simulink model "TEST"  (R2023a)
settings: Solver=ode1  StartTime=0.0  StopTime=tsim  FixedStep=CONTROL.Tm  RelTol=1e-3
undefined symbols (not defined in the file): Bm, J, MOTOR, tfalta, Tload, wini
libraries: simulink x2
settings Model: Creator=Usuario  LastModifiedBy=Usuario
settings DataIOCC: ReturnWorkspaceOutputs=off  TimeSaveName=time

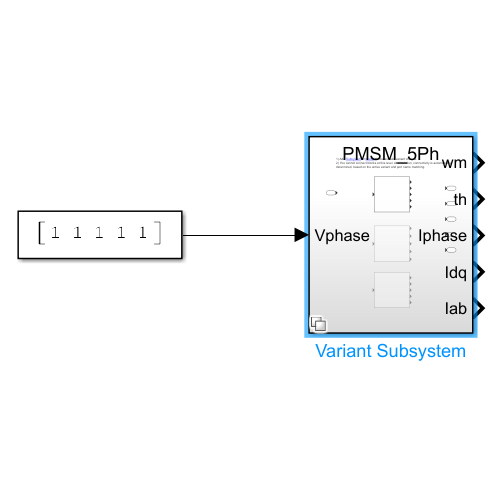
[thumbnail: Simulink's stored preview of the top-level diagram]
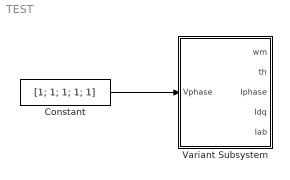
== system TEST ==
  Constant : Constant  Value=[1; 1; 1; 1; 1]
  Variant Subsystem : Subsystem  Variant=on
  wires:
  Constant/1 -> Variant Subsystem/1(Vphase)

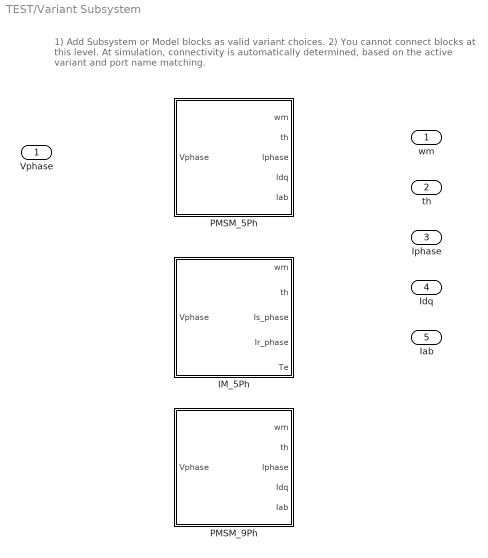
== system TEST/Variant Subsystem ==
  note: 1) Add Subsystem or Model blocks as valid variant choices.
      | 2) You cannot connect blocks at this level. At simulation, connectivity is automatically
      | determined, based on the active variant and port name matching.
  Vphase : Inport
  IM_5Ph : Subsystem  VariantControl=MOTOR.Index == 2
  PMSM_5Ph : Subsystem  VariantControl=MOTOR.Index == 1
  PMSM_9Ph : Subsystem  VariantControl=MOTOR.Index == 3
  wm : Outport
  th : Outport  Port=2
  Iphase : Outport  Port=3
  Idq : Outport  Port=4
  Iab : Outport  Port=5

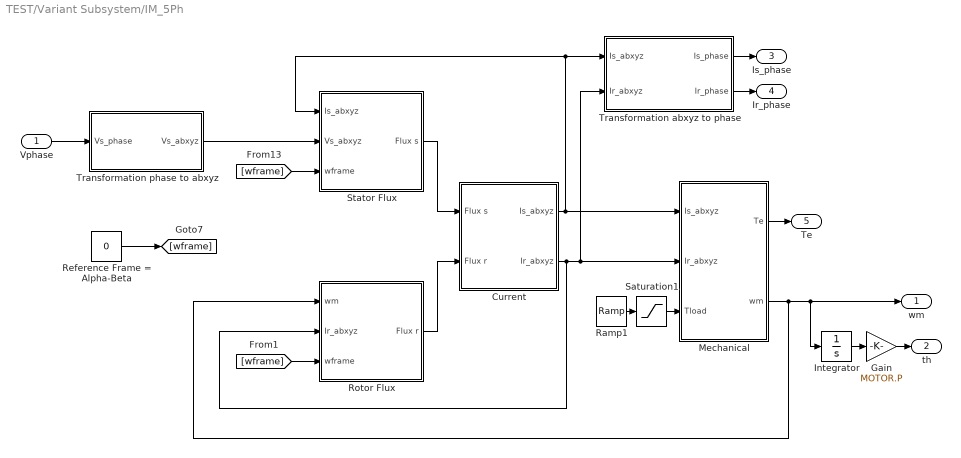
== system TEST/Variant Subsystem/IM_5Ph ==
  Vphase : Inport
  Current : Subsystem
  Gain : Gain  Gain=MOTOR.P
  Integrator : Integrator
  Mechanical : Subsystem
  Ramp1 : simulink/Sources/Ramp  slope=40*Tload  start=0  InitialOutput=0
  Reference Frame = Alpha-Beta : Constant  Value=0
  Rotor Flux : Subsystem
  Saturation1 : Saturate  UpperLimit=Tload  LowerLimit=0
  "Stator Flux " : Subsystem
  Transformation abxyz to phase : Subsystem
  Transformation phase to abxyz : Subsystem
  wm : Outport  VectorParamsAs1DForOutWhenUnconnected=off
  th : Outport  Port=2  VectorParamsAs1DForOutWhenUnconnected=off
  Is_phase : Outport  Port=3  VectorParamsAs1DForOutWhenUnconnected=off
  Ir_phase : Outport  Port=4  VectorParamsAs1DForOutWhenUnconnected=off
  Te : Outport  Port=5  VectorParamsAs1DForOutWhenUnconnected=off
  wires:
  Mechanical/1(Te) -> Te/1
  Transformation abxyz to phase/2(Ir_phase) -> Ir_phase/1
  [wframe] -> "Stator Flux "/3(wframe)
  Transformation phase to abxyz/1(Vs_abxyz) -> "Stator Flux "/2(Vs_abxyz)
  Ramp1/1 -> Saturation1/1
  Vphase/1 -> Transformation phase to abxyz/1(Vs_phase)
  Current/2(Ir_abxyz) -> Rotor Flux/2(Ir_abxyz), Transformation abxyz to phase/2(Ir_abxyz), Mechanical/2(Ir_abxyz)
  Current/1(Is_abxyz) -> Transformation abxyz to phase/1(Is_abxyz), "Stator Flux "/1(Is_abxyz), Mechanical/1(Is_abxyz)
  "Stator Flux "/1(Flux s) -> Current/1(Flux s)
  Reference Frame = Alpha-Beta/1 -> [wframe]
  Mechanical/2(wm) -> Integrator/1, wm/1, Rotor Flux/1(wm)
  Rotor Flux/1(Flux r) -> Current/2(Flux r)
  [wframe] -> Rotor Flux/3(wframe)
  Saturation1/1 -> Mechanical/3(Tload)
  Transformation abxyz to phase/1(Is_phase) -> Is_phase/1
  Integrator/1 -> Gain/1
  Gain/1 -> th/1

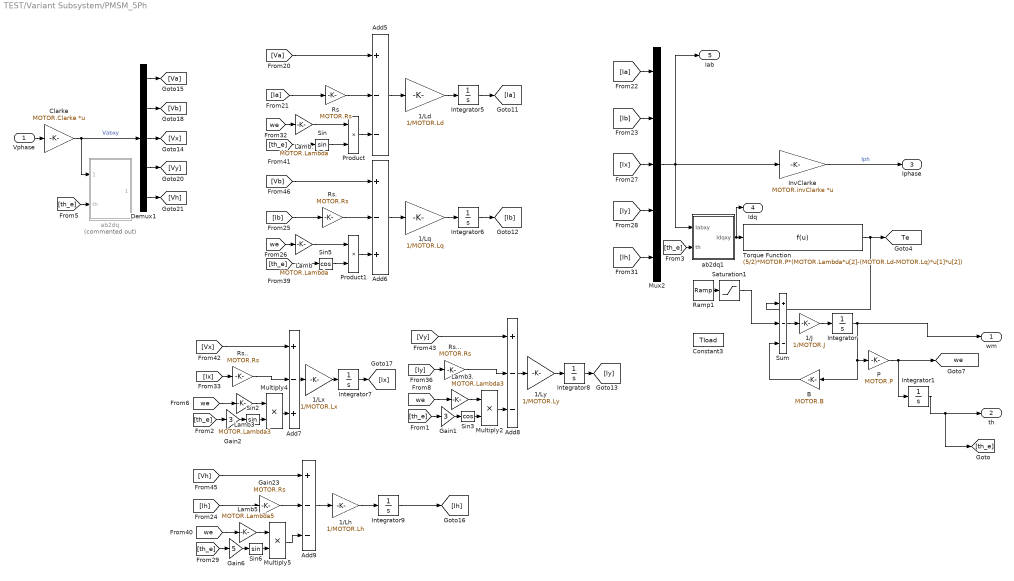
== system TEST/Variant Subsystem/PMSM_5Ph ==
  Vphase : Inport
  1/J : Gain  Gain=1/MOTOR.J
  1/Ld : Gain  Gain=1/MOTOR.Ld
  1/Lh : Gain  Gain=1/MOTOR.Lh
  1/Lq : Gain  Gain=1/MOTOR.Lq
  1/Lx : Gain  Gain=1/MOTOR.Lx
  1/Ly : Gain  Gain=1/MOTOR.Ly
  Add5 : Sum  Inputs=+--
  Add6 : Sum  Inputs=+-+
  Add7 : Sum  Inputs=+-+
  Add8 : Sum  Inputs=+--
  Add9 : Sum  Inputs=+--
  B : Gain  Gain=MOTOR.B
  Clarke : Gain  Gain=MOTOR.Clarke  Multiplication=Matrix(K*u)
  Constant3 : Constant  Value=Tload
  Demux1 : Demux  Outputs=5
  Gain1 : Gain  Gain=3
  Gain2 : Gain  Gain=3
  Gain23 : Gain  Gain=MOTOR.Rs
  Gain6 : Gain  Gain=5
  Integrator{,1,5..9} (7 alike) : Integrator
  InvClarke : Gain  Gain=MOTOR.invClarke  Multiplication=Matrix(K*u)
  Lamb : Gain  Gain=MOTOR.Lambda
  Lamb. : Gain  Gain=MOTOR.Lambda
  Lamb3 : Gain  Gain=MOTOR.Lambda3
  Lamb3. : Gain  Gain=MOTOR.Lambda3
  Lamb5 : Gain  Gain=MOTOR.Lambda5
  Multiply2 : Product
  Multiply4 : Product
  Multiply5 : Product
  Mux2 : Mux  Inputs=5
  P : Gain  Gain=MOTOR.P
  Product : Product
  Product1 : Product
  Ramp1 : simulink/Sources/Ramp  slope=40*Tload  start=0  InitialOutput=0
  Rs : Gain  Gain=MOTOR.Rs
  Rs. : Gain  Gain=MOTOR.Rs
  Rs.. : Gain  Gain=MOTOR.Rs
  Rs... : Gain  Gain=MOTOR.Rs
  Saturation1 : Saturate  UpperLimit=Tload  LowerLimit=0
  Sin : Trigonometry
  Sin2 : Trigonometry
  Sin3 : Trigonometry  Operator=cos
  Sin5 : Trigonometry  Operator=cos
  Sin6 : Trigonometry
  Sum : Sum  Inputs=+--
  Torque Function : Fcn  Expr=(5/2)*MOTOR.P*(MOTOR.Lambda*u[2]-(MOTOR.Ld-MOTOR.Lq)*u[1]*u[2])
  ab2dq : MATLAB Function  Commented=on  TreatAsAtomicUnit=on
  ab2dq1 : MATLAB Function  TreatAsAtomicUnit=on
  wm : Outport
  th : Outport  Port=2
  Iphase : Outport  Port=3
  Idq : Outport  Port=4
  Iab : Outport  Port=5
  tag scope: Te=global, we=global
  wires:
  Gain6/1 -> Sin6/1
  [we] -> Lamb5/1
  Ramp1/1 -> Saturation1/1
  Sin6/1 -> Multiply5/2
  [Va] -> Add5/1
  Lamb5/1 -> Multiply5/1
  Gain1/1 -> Sin3/1
  Lamb3./1 -> Multiply2/1
  1/Lq/1 -> Integrator6/1
  Add8/1 -> 1/Ly/1
  [th_e] -> Gain1/1
  [th_e] -> Gain6/1
  [we] -> Lamb3./1
  Add6/1 -> 1/Lq/1
  [Ix] -> Mux2/3
  Sin/1 -> Product/2
  [th_e] -> Sin/1
  Vphase/1 -> Clarke/1
  1/Ly/1 -> Integrator8/1
  [th_e] -> Sin5/1
  Integrator8/1 -> [Iy]
  Multiply2/1 -> Add8/3
  [we] -> Lamb/1
  Demux1/3 -> [Vx]
  Sin3/1 -> Multiply2/2
  Lamb/1 -> Product1/1
  Sin5/1 -> Product1/2
  ab2dq1/1(Idqxy) -> Torque Function/1, Idq/1
  Rs/1 -> Add5/2
  Rs.../1 -> Add8/2
  Integrator5/1 -> [Ia]
  [Ih] -> Gain23/1
  [we] -> Lamb./1
  [th_e] -> ab2dq/2(th)
  [th_e] -> ab2dq1/2(th)
  [Ib] -> Rs./1
  Rs../1 -> Add7/2
  B/1 -> Sum/3
  InvClarke/1 -> Iphase/1  "Iph"
  Product/1 -> Add5/3
  [Vb] -> Add6/1
  1/Lh/1 -> Integrator9/1
  [Ia] -> Rs/1
  Add9/1 -> 1/Lh/1
  Demux1/2 -> [Vb]
  [Vh] -> Add9/1
  Integrator/1 -> P/1, B/1, wm/1
  Torque Function/1 -> [Te], Sum/1
  Saturation1/1 -> Sum/2
  Integrator1/1 -> [th_e], th/1
  1/Lx/1 -> Integrator7/1
  Sum/1 -> 1/J/1
  Clarke/1 -> Demux1/1, ab2dq/1(Vabxy)  "Vabxy"
  [Ia] -> Mux2/1
  Lamb3/1 -> Multiply4/1
  [Ib] -> Mux2/2
  Add5/1 -> 1/Ld/1
  [Ih] -> Mux2/5
  Product1/1 -> Add6/3
  Add7/1 -> 1/Lx/1
  Rs./1 -> Add6/2
  Integrator9/1 -> [Ih]
  [th_e] -> Gain2/1
  [Iy] -> Mux2/4
  1/Ld/1 -> Integrator5/1
  1/J/1 -> Integrator/1
  Integrator7/1 -> [Ix]
  Demux1/5 -> [Vh]
  Gain23/1 -> Add9/2
  Integrator6/1 -> [Ib]
  Demux1/1 -> [Va]
  P/1 -> Integrator1/1, [we]
  [Iy] -> Rs.../1
  Mux2/1 -> InvClarke/1, ab2dq1/1(Iabxy), Iab/1
  Lamb./1 -> Product/1
  [Vy] -> Add8/1
  Gain2/1 -> Sin2/1
  Demux1/4 -> [Vy]
  Multiply5/1 -> Add9/3
  [we] -> Lamb3/1
  [Ix] -> Rs../1
  [Vx] -> Add7/1
  Multiply4/1 -> Add7/3
  Sin2/1 -> Multiply4/2

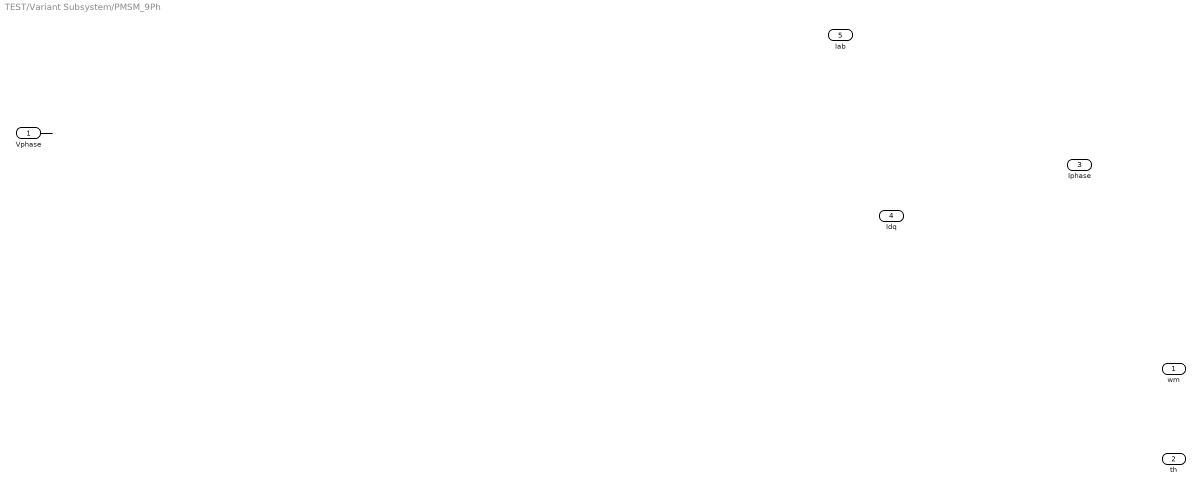
== system TEST/Variant Subsystem/PMSM_9Ph ==
  Vphase : Inport
  wm : Outport
  th : Outport  Port=2
  Iphase : Outport  Port=3
  Idq : Outport  Port=4
  Iab : Outport  Port=5
  wires:
  Vphase/1 -> ?

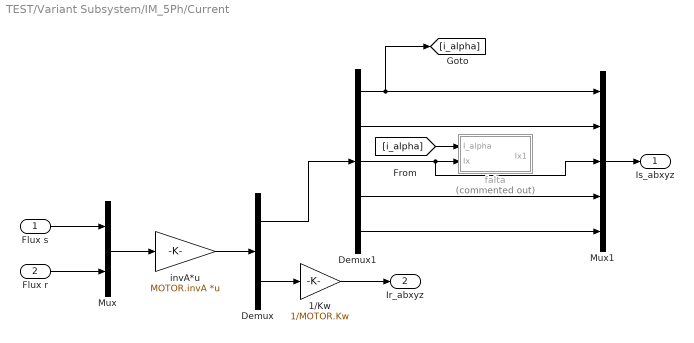
== system TEST/Variant Subsystem/IM_5Ph/Current ==
  Flux s : Inport
  Flux r : Inport  Port=2
  1/Kw : Gain  Gain=1/MOTOR.Kw
  Demux : Demux  Outputs=2
  Demux1 : Demux  Outputs=5
  Mux : Mux  Inputs=2
  Mux1 : Mux  Inputs=5
  falta : Subsystem  Commented=on
  invA*u : Gain  Gain=MOTOR.invA  Multiplication=Matrix(K*u)
  Is_abxyz : Outport  VectorParamsAs1DForOutWhenUnconnected=off
  Ir_abxyz : Outport  Port=2  VectorParamsAs1DForOutWhenUnconnected=off
  wires:
  Flux s/1 -> Mux/1
  Flux r/1 -> Mux/2
  Mux/1 -> invA*u/1
  invA*u/1 -> Demux/1
  Demux/2 -> 1/Kw/1
  1/Kw/1 -> Ir_abxyz/1
  Demux1/1 -> [i_alpha], Mux1/1
  Demux1/2 -> Mux1/2
  Demux1/4 -> Mux1/4
  Demux1/5 -> Mux1/5
  Mux1/1 -> Is_abxyz/1
  Demux/1 -> Demux1/1
  [i_alpha] -> falta/1(I_alpha)
  Demux1/3 -> Mux1/3, falta/2(Ix)

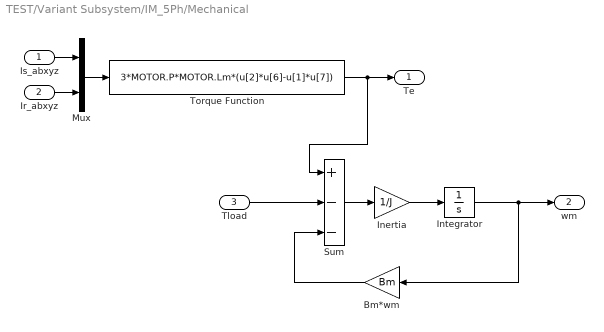
== system TEST/Variant Subsystem/IM_5Ph/Mechanical ==
  Is_abxyz : Inport
  Ir_abxyz : Inport  Port=2
  Tload : Inport  Port=3
  Bm*wm : Gain  Gain=Bm
  Inertia : Gain  Gain=1/J
  Integrator : Integrator  InitialCondition=wini
  Mux : Mux  Inputs=2
  Sum : Sum  Inputs=+--
  Torque Function : Fcn  Expr=3*MOTOR.P*MOTOR.Lm*(u[2]*u[6]-u[1]*u[7])
  Te : Outport  VectorParamsAs1DForOutWhenUnconnected=off
  wm : Outport  Port=2  VectorParamsAs1DForOutWhenUnconnected=off
  wires:
  Tload/1 -> Sum/2
  Sum/1 -> Inertia/1
  Inertia/1 -> Integrator/1
  Bm*wm/1 -> Sum/3
  Integrator/1 -> wm/1, Bm*wm/1
  Is_abxyz/1 -> Mux/1
  Ir_abxyz/1 -> Mux/2
  Mux/1 -> Torque Function/1
  Torque Function/1 -> Sum/1, Te/1

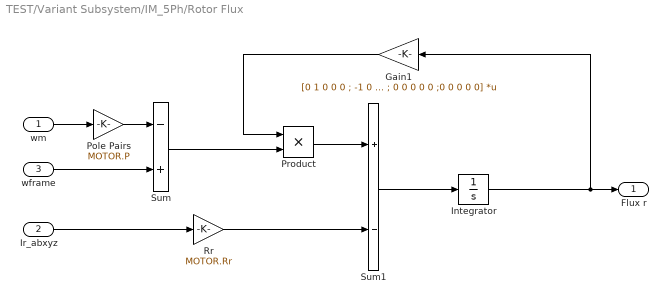
== system TEST/Variant Subsystem/IM_5Ph/Rotor Flux ==
  wm : Inport
  Ir_abxyz : Inport  Port=2
  wframe : Inport  Port=3
  Gain1 : Gain  Gain=[0 1 0 0 0 ; -1 0 0 0 0 ; 0 0 0 0 0 ; 0 0 0 0 0 ;0 0 0 0 0]  Multiplication=Matrix(K*u)
  Integrator : Integrator
  Pole Pairs : Gain  Gain=MOTOR.P
  Product : Product  RndMeth=Zero
  Rr : Gain  Gain=MOTOR.Rr
  Sum : Sum  Inputs=-+
  Sum1 : Sum  Inputs=+-
  Flux r : Outport  VectorParamsAs1DForOutWhenUnconnected=off
  wires:
  Ir_abxyz/1 -> Rr/1
  Product/1 -> Sum1/1
  Rr/1 -> Sum1/2
  wframe/1 -> Sum/2
  Sum1/1 -> Integrator/1
  Integrator/1 -> Flux r/1, Gain1/1
  Gain1/1 -> Product/1
  wm/1 -> Pole Pairs/1
  Pole Pairs/1 -> Sum/1
  Sum/1 -> Product/2

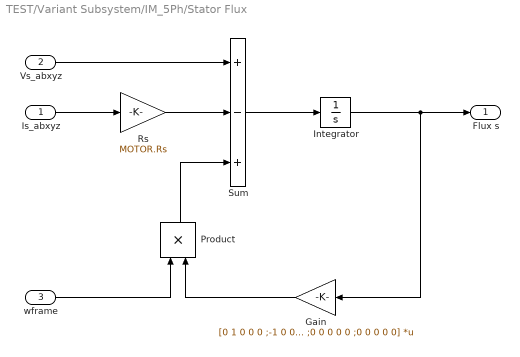
== system TEST/Variant Subsystem/IM_5Ph/Stator Flux  ==
  Is_abxyz : Inport
  Vs_abxyz : Inport  Port=2
  wframe : Inport  Port=3
  Gain : Gain  Gain=[0 1 0 0 0 ;-1 0 0 0 0 ;0 0 0 0 0 ;0 0 0 0 0 ;0 0 0 0 0]  Multiplication=Matrix(K*u)
  Integrator : Integrator
  Product : Product  RndMeth=Zero
  Rs : Gain  Gain=MOTOR.Rs
  Sum : Sum  Inputs=+-+
  Flux s : Outport  VectorParamsAs1DForOutWhenUnconnected=off
  wires:
  Rs/1 -> Sum/2
  Sum/1 -> Integrator/1
  Integrator/1 -> Gain/1, Flux s/1
  Is_abxyz/1 -> Rs/1
  Vs_abxyz/1 -> Sum/1
  Product/1 -> Sum/3
  wframe/1 -> Product/1
  Gain/1 -> Product/2

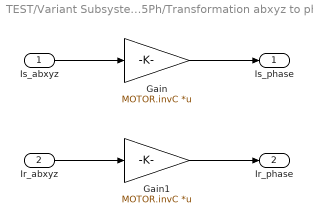
== system TEST/Variant Subsystem/IM_5Ph/Transformation abxyz to phase ==
  Is_abxyz : Inport
  Ir_abxyz : Inport  Port=2
  Gain : Gain  Gain=MOTOR.invC  Multiplication=Matrix(K*u)
  Gain1 : Gain  Gain=MOTOR.invC  Multiplication=Matrix(K*u)
  Is_phase : Outport  VectorParamsAs1DForOutWhenUnconnected=off
  Ir_phase : Outport  Port=2  VectorParamsAs1DForOutWhenUnconnected=off
  wires:
  Is_abxyz/1 -> Gain/1
  Gain/1 -> Is_phase/1
  Ir_abxyz/1 -> Gain1/1
  Gain1/1 -> Ir_phase/1

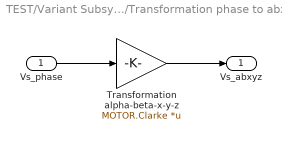
== system TEST/Variant Subsystem/IM_5Ph/Transformation phase to abxyz ==
  Vs_phase : Inport
  Transformation alpha-beta-x-y-z : Gain  Gain=MOTOR.Clarke  Multiplication=Matrix(K*u)
  Vs_abxyz : Outport  VectorParamsAs1DForOutWhenUnconnected=off
  wires:
  Transformation alpha-beta-x-y-z/1 -> Vs_abxyz/1
  Vs_phase/1 -> Transformation alpha-beta-x-y-z/1

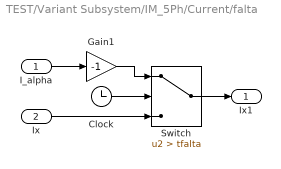
== system TEST/Variant Subsystem/IM_5Ph/Current/falta ==
  I_alpha : Inport
  Ix : Inport  Port=2
  Clock : Clock
  Gain1 : Gain  Gain=-1
  Switch : Switch  Criteria=u2 > Threshold  Threshold=tfalta  SaturateOnIntegerOverflow=off  InputSameDT=off
  Ix1 : Outport  VectorParamsAs1DForOutWhenUnconnected=off
  wires:
  Ix/1 -> Switch/3
  Switch/1 -> Ix1/1
  Clock/1 -> Switch/2
  I_alpha/1 -> Gain1/1
  Gain1/1 -> Switch/1

== matlab function TEST/Variant Subsystem/PMSM_5Ph/ab2dq ==
  data: Vabxy input; Vdqxy output; th input
 function Vdqxy = Park(Vabxy,th)

% Mp= [ cos(th)   sin(th)           0         0          0
%      -sin(th)   cos(th)           0         0          0 
%          0           0        cos(3*th)   -sin(3*th)   0
%          0           0        sin(3*th)    cos(3*th)   0
%          0           0            0         0          1];
Vdqxy = zeros(5,1);
Mp= [ cos(th)   sin(th)  0  0  0
     -sin(th)   cos(th)  0  0  0 
         0           0   1  0  0
         0           0   0  1  0
         0           0   0  0  1];

Vdqxy = Mp*Vabxy;
end

== matlab function TEST/Variant Subsystem/PMSM_5Ph/ab2dq1 ==
  data: Iabxy input; Idqxy output; th input
 function Idqxy = Park(Iabxy,th)

% Mp= [ cos(th)   sin(th)           0         0          0
%      -sin(th)   cos(th)           0         0          0 
%          0           0        cos(3*th)   -sin(3*th)   0
%          0           0        sin(3*th)    cos(3*th)   0
%          0           0            0         0          1];
Idqxy = zeros(5,1);
Mp= [ cos(th)   sin(th)  0  0  0
     -sin(th)   cos(th)  0  0  0 
         0           0   1  0  0
         0           0   0  1  0
         0           0   0  0  1];

Idqxy = Mp*Iabxy;
end
